simulink model "hdlcoder_fft32_eml"  (R2026a)
settings: Solver=FixedStepDiscrete  FixedStep=1  EnableMultiTasking=on
libraries: dspxfrm3 x1
settings Model: Creator=The MathWorks, Inc.  LastModifiedBy=The MathWorks, Inc.
settings OptimizationCC: InitFltsAndDblsToZero=on
settings DebuggingCC: SaveWithParameterizedLinksMsg=none  UnderspecifiedInitializationDetection=Classic  MultiTaskDSMMsg=warning  MultiTaskCondExecSysMsg=none
settings HardwareCC: ProdHWDeviceType=32-bit Generic  TargetHWDeviceType=32-bit Generic
settings GRTTargetCC: TargetFcnLib=ansi_tfl_tmw.mat  CombineOutputUpdateFcns=off  GRTInterface=on

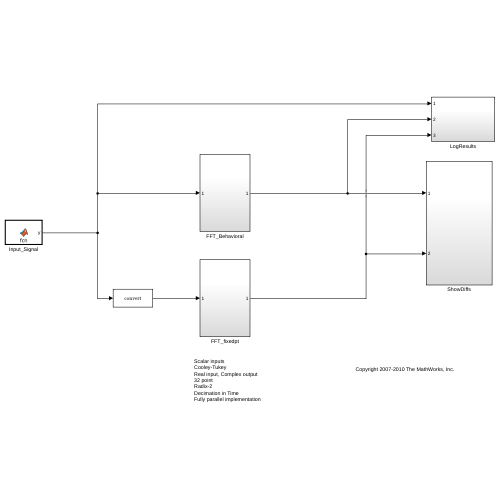
[thumbnail: Simulink's stored preview of the top-level diagram]
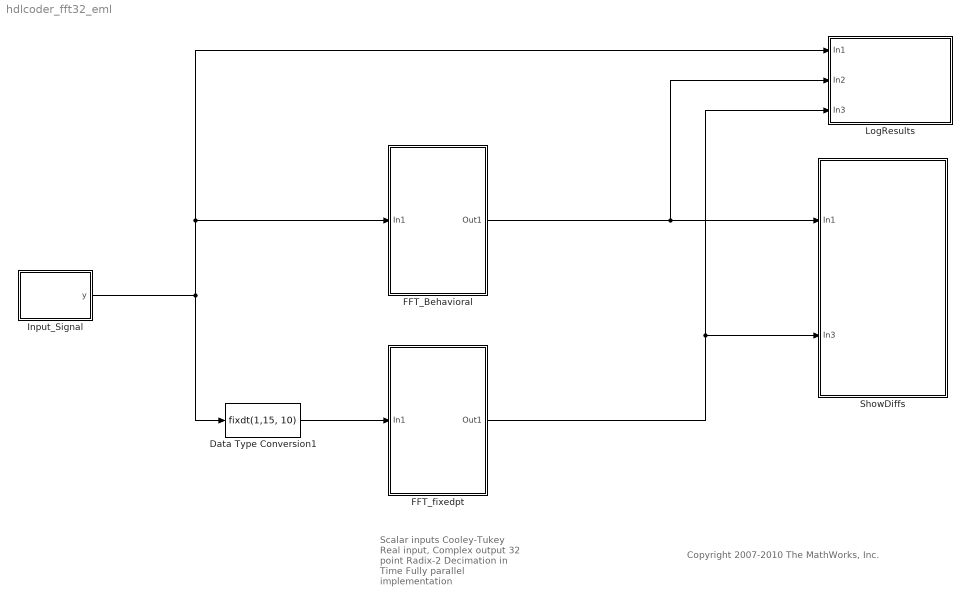
== system hdlcoder_fft32_eml ==
  note: Scalar inputs
      | Cooley-Tukey
      | Real input, Complex output
      | 32 point
      | Radix-2
      | Decimation in Time
      | Fully parallel implementation
  note: Copyright 2007-2010 The MathWorks, Inc.
  Data Type Conversion1 : DataTypeConversion  OutDataTypeStr=fixdt(1,15, 10)  SaturateOnIntegerOverflow=off  RndMeth=Floor
  FFT_Behavioral : Subsystem
  FFT_fixedpt : Subsystem
  Input_Signal : MATLAB Function  TreatAsAtomicUnit=on
  LogResults : Subsystem
  ShowDiffs : Subsystem
  wires:
  FFT_Behavioral/1(Out1) -> ShowDiffs/1(In1), LogResults/2(In2)
  Data Type Conversion1/1 -> FFT_fixedpt/1(In1)
  FFT_fixedpt/1(Out1) -> ShowDiffs/2(In3), LogResults/3(In3)
  Input_Signal/1(y) -> FFT_Behavioral/1(In1), LogResults/1(In1), Data Type Conversion1/1

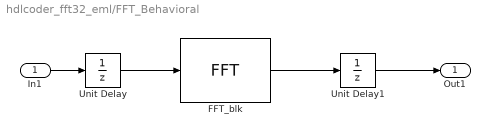
== system hdlcoder_fft32_eml/FFT_Behavioral ==
  In1 : Inport
  FFT_blk : dspxfrm3/FFT  FFTImplementation=Auto  CompMethod=Table lookup  TableOpt=HYBRID  TableOptActive=Speed  BitRevOrder=off  Normalize=off  InheritFFTLength=on  FFTLength=64  WrapInput=on  roundingMode=Floor  overflowMode=off  firstCoeffDataTypeStr=Inherit: Same word length as input  firstCoeffLastDataTypeStr=Inherit: Same word length as input  outputMin=[]  outputMax=[]
  Unit Delay : UnitDelay
  Unit Delay1 : UnitDelay
  Out1 : Outport
  wires:
  Unit Delay/1 -> FFT_blk/1
  In1/1 -> Unit Delay/1
  FFT_blk/1 -> Unit Delay1/1
  Unit Delay1/1 -> Out1/1

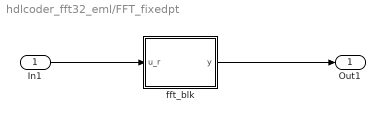
== system hdlcoder_fft32_eml/FFT_fixedpt ==
  In1 : Inport
  fft_blk : MATLAB Function  TreatAsAtomicUnit=on
  Out1 : Outport
  wires:
  In1/1 -> fft_blk/1(u_r)
  fft_blk/1(y) -> Out1/1

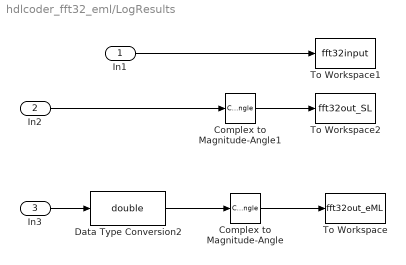
== system hdlcoder_fft32_eml/LogResults ==
  In1 : Inport
  In2 : Inport  Port=2
  In3 : Inport  Port=3
  Complex to Magnitude-Angle : ComplexToMagnitudeAngle  Output=Magnitude
  Complex to Magnitude-Angle1 : ComplexToMagnitudeAngle  Output=Magnitude
  Data Type Conversion2 : DataTypeConversion  OutDataTypeStr=double  SaturateOnIntegerOverflow=off  RndMeth=Floor
  To Workspace : ToWorkspace  VariableName=fft32out_eML  SampleTime=1
      settings: MaxDataPoints=1
  To Workspace1 : ToWorkspace  VariableName=fft32input  SampleTime=1
      settings: MaxDataPoints=1
  To Workspace2 : ToWorkspace  VariableName=fft32out_SL  SampleTime=1
      settings: MaxDataPoints=1
  wires:
  Complex to Magnitude-Angle/1 -> To Workspace/1
  Complex to Magnitude-Angle1/1 -> To Workspace2/1
  Data Type Conversion2/1 -> Complex to Magnitude-Angle/1
  In1/1 -> To Workspace1/1
  In2/1 -> Complex to Magnitude-Angle1/1
  In3/1 -> Data Type Conversion2/1

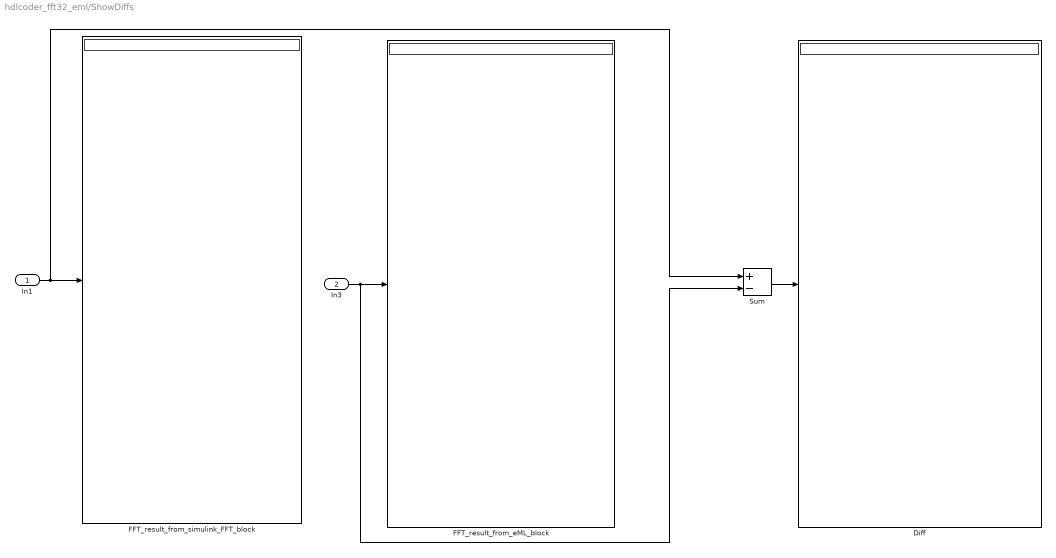
== system hdlcoder_fft32_eml/ShowDiffs ==
  In1 : Inport
  In3 : Inport  Port=2
  Diff : Display
  FFT_result_from_eML_block : Display
  FFT_result_from_simulink_FFT_block : Display
  Sum : Sum  Inputs=+-
  wires:
  In1/1 -> FFT_result_from_simulink_FFT_block/1, Sum/1
  In3/1 -> FFT_result_from_eML_block/1, Sum/2
  Sum/1 -> Diff/1

== matlab function hdlcoder_fft32_eml/FFT_fixedpt/fft_blk ==
  settings: fimath=|
      | fimath(...
      | 'RoundMode', 'floor',...
      | 'OverflowMode', 'wrap',...
      | 'ProductMode', 'FullPrecision', 'ProductWordLength', 32,...
      | 'SumMode', 'FullPrecision', 'SumWordLength', 32,...
      | 'CastBeforeSum', true)
  data: u_r input size=32; y output
function y  = fcn(u_r)
% 32point FFT
% Real input and Complex output
% Cooley-Tukey
% Radix-2
% Decimation in Time

% N point FFT involves N/2 stages.
% 


N = 32;

%reverse input order
bu_r = bitrevorder_hdl(u_r);
bu_i = fi(zeros(32, 1), numerictype(u_r), fimath(u_r));

u = complex(bu_r, bu_i);

y = fft32(N, u);

end

%fft32
function x = fft32(N, u)

nt = numerictype(u);
fm = fimath(u);

x = complex(fi(zeros(32,1), nt, fm));

tu1 = fft16(N, u(1:16));
tu2 = fft16(N, u(17:32));

for i=1:16
    tw = twf(N, (i-1));
    twu = hdlfi_mul(tu2(i), tw);
    [x(i), x(i+16)] = bfly2(tu1(i), twu);
end
end

%fft16
function x = fft16(N, u)

nt = numerictype(u);
fm = fimath(u);

x = complex(fi(zeros(16,1), nt, fm));

tu1 = fft8(N, u(1:8));
tu2 = fft8(N, u(9:16));

for i=1:8
    tw = twf(N, (i-1)*2);
    twu = hdlfi_mul(tu2(i) , tw);
    [x(i), x(i+8)] = bfly2(tu1(i), twu);
end
end

%fft8
function x = fft8(N, u)

nt = numerictype(u);
fm = fimath(u);

x = complex(fi(zeros(8,1), nt, fm));

tu1 = fft4(N, u(1:4));
tu2 = fft4(N, u(5:8));

for i=1:4
    tw = twf(N, (i-1)*4);
    twu = hdlfi_mul(tu2(i) , tw);
    [x(i), x(i+4)] = bfly2(tu1(i), twu);
end
end

%fft4
function x = fft4(N, u)

nt = numerictype(u);
fm = fimath(u);

x = complex(fi(zeros(4,1), nt, fm));

tu1 = complex(fi(zeros(2,1), nt, fm));
tu2 = complex(fi(zeros(2,1), nt, fm));

[tu1(1), tu1(2)] = bfly2(u(1), u(2));
[tu2(1), tu2(2)] = bfly2(u(3), u(4));

% typical butterfly structure in an FFT
%
%    u0 --------------> tu0
%               \   /
%                \ /
%                 x
%                / \
%               /   \
%   u1 ---------------> tu1
%        tw         

for i=1:2
    tw = twf(N, (i-1)*8);
    twu = hdlfi_mul(tu2(i) , tw);
    [x(i), x(i+2)] = bfly2(tu1(i), twu);
end
end


function [x, y] = bfly2(u, v)
%% Two element butterfly
% use sum_fm and sum_nt to clamp the result of addition

sum_fm = fimath(...
'RoundMode', 'floor',...
'OverflowMode', 'wrap',...
'ProductMode', 'FullPrecision', 'ProductWordLength', 32,...
'SumMode', 'FullPrecision', 'SumWordLength', 32,...
'CastBeforeSum', true);

sum_nt = numerictype(1, 15, 10);

x = fi(u + v, sum_nt, sum_fm);
y = fi(u - v, sum_nt, sum_fm);

end

function out = hdlfi_mul(in1, in2)
%% Complex fi multiplication
% use mul_fm and mul_nt to clamp the result of multiplication

mul_fm = fimath(...
'RoundMode', 'floor',...
'OverflowMode', 'wrap',...
'ProductMode', 'FullPrecision', 'ProductWordLength', 32,...
'SumMode', 'FullPrecision', 'SumWordLength', 32,...
'CastBeforeSum', true);

mul_nt = numerictype(1,15, 10);

out = fi(in1 * in2, mul_nt, mul_fm);

end

function W = twf(N, k)
%% complex roots of unity (N=32)
%W = exp(-2*pi*1i*k/N)

twf_fm = fimath(...
'RoundMode', 'floor',...
'OverflowMode', 'wrap',...
'ProductMode', 'FullPrecision', 'ProductWordLength', 32,...
'SumMode', 'FullPrecision', 'SumWordLength', 32,...
'CastBeforeSum', true);

twf_nt = numerictype(1,15, 10);


persistent w_N
if isempty(w_N)
    w_N = fi(exp(-2*pi*1i*(0:(N-1))/N).', twf_nt, twf_fm);
end
W = w_N(k+1);

end


function y = bitrevorder_hdl(u) 
% This function reorders elements of 'u' by computing new index positions 
% that have the bit reversed values of the original index position

N = uint32(length(u));

if bitand(N, 1) ~= 0
    error('invalid input, input length must be even');
end

idx_vec = uint32(0:N-1);
len_pow2 = log2(length(u));

fi_idx_vec = fi(idx_vec, 0, len_pow2, 0);

for ii=1:length(fi_idx_vec)  
    fi_idx_vec(ii) = bitreverse(fi_idx_vec(ii));
end

brev_idx = int32(fi_idx_vec)+1;
y = u(brev_idx);

end

function y = bitreverse(u)
t = u;

nt = numerictype(u);
nt2 = floor(nt.WordLength/2);

for ii=1:nt2
    a = bitget(u, ii);
    b = bitget(u, nt.WordLength-ii+1);
    t = bitset(t, ii, b);
    t = bitset(t, nt.WordLength-ii+1, a);
end

y = t;
end

== matlab function hdlcoder_fft32_eml/Input_Signal ==
  data: y output
function y = fcn
%#codegen

% Fs = 4;                                     % Sampling frequency in Hz
% t  = (0:31)/Fs;                          % Time vector
% f0 = .2; f1 = .5;                           % Frequencies, in Hz
% y = (cos(2*pi*f0*t) + 0.55*cos(2*pi*f1*t))';


y = [1.5500
    1.3400
    0.8090
    0.1989
   -0.2410
   -0.3889
   -0.3090
   -0.1989
   -0.2590
   -0.5621
   -1.0000
   -1.3400
   -1.3590
   -0.9767
   -0.3090
    0.3889
    0.8590
    0.9767
    0.8090
    0.5621
    0.4500
    0.5621
    0.8090
    0.9767
    0.8590
    0.3889
   -0.3090
   -0.9767
   -1.3590
   -1.3400
   -1.0000
   -0.5621];
